simulink model "lateralb747"  (R2024b)
settings: Solver=ode4  StartTime=0.0  StopTime=inf  FixedStep=0.001  RelTol=1e-3
values from neighbouring files (symbols this model uses):
  alpha_init = p.alpharef    [b747lateral.m]
  theta_init = alpha_init    [b747lateral.m]
  V_init = 67.394444    [b747lateral.m]
undefined symbols (not defined in the file or in its folder): p
libraries: simulink_extras x4
settings Model: Creator=adasu  LastModifiedBy=adasu

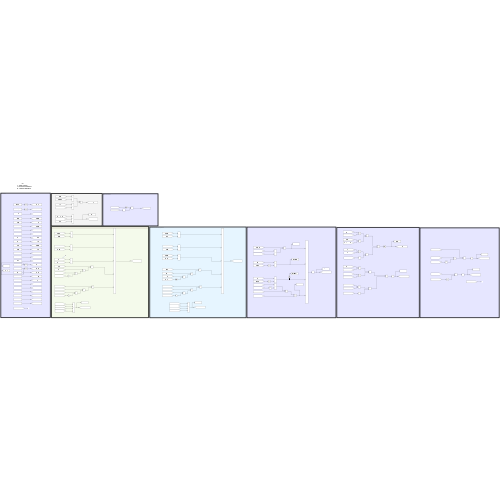
[thumbnail: Simulink's stored preview of the top-level diagram]
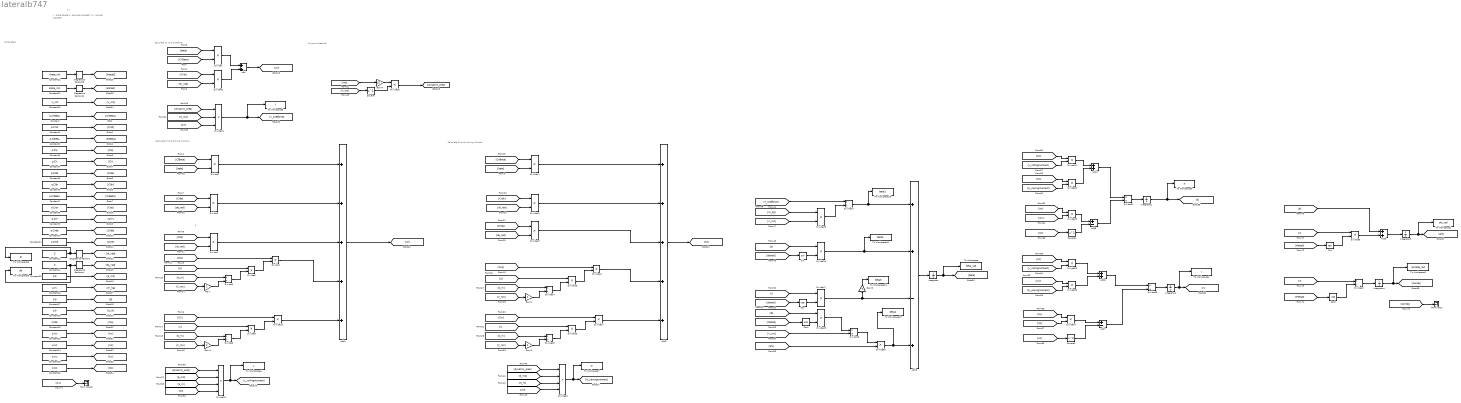
== system lateralb747 ==
  note: Dynamic Pressure
  note: Calculate Cn and Yawing Moment
  note: Calculate Cl and Rolling Moment
  note: Calculate CY and Sideforce
  note: !!!!!
  note: Parameters
  note: Y : SIDE FORCE
      | L : ROLLING MOMENT
      | N : YAWING MOMENT
  note: 0
  Add{,4,6,8} (4 alike) : Sum
  Add1 : Sum  Inputs=5
  Add2 : Sum  Inputs=5
  Add3 : Sum  Inputs=++-+
  Add5 : Sum  Inputs=+-
  Add7 : Sum  Inputs=+-
  Constant : Constant  Value=p.CYBeta
  Constant1 : Constant  Value=p.CYdr
  Constant10 : Constant  Value=p.Cnda
  Constant11 : Constant  Value=p.Cndr
  Constant12 : Constant  Value=5
  Constant14 : Constant  Value=0
  Constant15 : Constant  Value=p.S
  Constant16 : Constant  Value=p.m
  Constant17 : Constant  Value=p.g
  Constant18 : Constant  Value=p.b
  Constant19 : Constant  Value=1.225
  Constant2 : Constant  Value=p.ClBeta
  Constant20 : Constant  Value=V_init
  Constant21 : Constant  Value=alpha_init
  Constant22 : Constant  Value=theta_init
  Constant23 : Constant  Value=p.Ixx
  Constant24 : Constant  Value=p.Ixz
  Constant25 : Constant  Value=p.Iyy
  Constant26 : Constant  Value=p.Izz
  Constant3 : Constant  Value=p.Clp
  Constant4 : Constant  Value=p.Clr
  Constant5 : Constant  Value=p.Clda
  Constant6 : Constant  Value=p.Cldr
  Constant7 : Constant  Value=p.CnBeta
  Constant8 : Constant  Value=p.Cnp
  Constant9 : Constant  Value=p.Cnr
  Cos : Trigonometry  Operator=cos
  Cos1 : Trigonometry  Operator=cos
  Cos2 : Trigonometry  Operator=cos
  Degrees to Radians{,1..3} (4 alike) : simulink_extras/Transformations/Degrees to Radians
  Divide{1..4,6..7,9..13,15..17,19..20,25..28,30..33,35..37,39,41} (29 alike) : Product  Inputs=**
  Divide{5,8,14,18,24,29,34,38,40} (9 alike) : Product  Inputs=*/
  Divide21 : Product  Inputs=***
  Divide22 : Product  Inputs=****
  Divide23 : Product  Inputs=****
  Gain{,1..3} (4 alike) : Gain  Gain=2
  Gain4 : Gain  Gain=1/2
  Gain5 : Gain  Gain=-1
  Integrator{,1..4} (5 alike) : Integrator
  Sin : Trigonometry
  Square : Math  Operator=square
  Square1 : Math  Operator=square
  Square2 : Math  Operator=square
  Tan : Trigonometry  Operator=tan
  Terminator : Terminator
  Terminator2 : Terminator
  To Workspace : ToWorkspace  VariableName=beta_rad  SaveFormat=Timeseries  SampleTime=-1
  To Workspace1 : ToWorkspace  VariableName=phi_rad  SaveFormat=Timeseries  SampleTime=-1
  To Workspace10 : ToWorkspace  VariableName=beta1  SaveFormat=Timeseries  SampleTime=-1
  To Workspace11 : ToWorkspace  VariableName=beta2  SaveFormat=Timeseries  SampleTime=-1
  To Workspace12 : ToWorkspace  VariableName=beta3  SaveFormat=Timeseries  SampleTime=-1
  To Workspace13 : ToWorkspace  VariableName=beta4  SaveFormat=Timeseries  SampleTime=-1
  To Workspace2 : ToWorkspace  VariableName=lambda_rad  SaveFormat=Timeseries  SampleTime=-1
  To Workspace3 : ToWorkspace  VariableName=p  SaveFormat=Timeseries  SampleTime=-1
  To Workspace4 : ToWorkspace  VariableName=r  SaveFormat=Timeseries  SampleTime=-1
  To Workspace5 : ToWorkspace  VariableName=Y  SaveFormat=Timeseries  SampleTime=-1
  To Workspace6 : ToWorkspace  VariableName=L  SaveFormat=Timeseries  SampleTime=-1
  To Workspace7 : ToWorkspace  VariableName=N  SaveFormat=Timeseries  SampleTime=-1
  To Workspace8 : ToWorkspace  VariableName=dr  SaveFormat=Timeseries  SampleTime=-1
  To Workspace9 : ToWorkspace  VariableName=da  SaveFormat=Timeseries  SampleTime=-1
  wires:
  Constant/1 -> [CYBeta]
  Constant1/1 -> [CYdr]
  Constant2/1 -> [ClBeta]
  Constant3/1 -> [Clp]
  Constant4/1 -> [Clr]
  Constant5/1 -> [Clda]
  Constant6/1 -> [Cldr]
  Constant7/1 -> [CnBeta]
  Constant8/1 -> [Cnp]
  Constant9/1 -> [Cnr]
  Constant10/1 -> [Cnda]
  Constant11/1 -> [Cndr]
  Constant12/1 -> To Workspace8/1, Degrees to Radians/1
  Degrees to Radians/1 -> [dr_rad]
  [beta] -> Divide1/1
  [CYBeta] -> Divide1/2
  Divide1/1 -> Add/1
  Divide41/1 -> Add/2
  Add/1 -> [CY]
  Degrees to Radians1/1 -> [da_rad]
  Constant14/1 -> To Workspace9/1, Degrees to Radians1/1
  Constant15/1 -> [S_m2]
  Constant16/1 -> [m_kg]
  Constant17/1 -> [g]
  Constant18/1 -> [b_m]
  Constant19/1 -> [rho]
  Gain4/1 -> Divide20/1
  Divide20/1 -> [dynamic_pres]
  Square/1 -> Divide20/2
  [V_ms] -> Square/1
  [rho] -> Gain4/1
  [S_m2] -> Divide21/2
  [dynamic_pres] -> Divide21/1
  [CY] -> Divide21/3
  Divide21/1 -> To Workspace5/1, [Y_sideforce]
  Divide22/1 -> To Workspace6/1, [L_rollingmoment]
  [dynamic_pres] -> Divide22/1
  [S_m2] -> Divide22/2
  [b_m] -> Divide22/3
  [Cl] -> Divide22/4
  [Cn] -> Divide23/4
  [b_m] -> Divide23/3
  [S_m2] -> Divide23/2
  [dynamic_pres] -> Divide23/1
  Divide23/1 -> To Workspace7/1, [N_yawingmoment]
  [Y_sideforce] -> Divide24/1
  Divide25/1 -> Divide24/2
  Constant21/1 -> Degrees to Radians2/1
  Degrees to Radians2/1 -> [alpha0]
  [alpha0] -> Sin/1
  Sin/1 -> Divide26/2
  [alpha0] -> Cos/1
  Degrees to Radians3/1 -> [theta0]
  Constant22/1 -> Degrees to Radians3/1
  [theta0] -> Cos1/1
  Divide28/1 -> Divide29/1
  [V_ms] -> Divide29/2
  [phi] -> Divide30/2
  Divide29/1 -> Divide30/1
  Divide24/1 -> To Workspace10/1, Add3/1
  Divide26/1 -> To Workspace11/1, Add3/2
  Divide27/1 -> Gain5/1, Add3/3
  Divide30/1 -> To Workspace13/1, Add3/4
  Add3/1 -> Integrator/1
  Integrator/1 -> To Workspace/1, [beta]
  Constant23/1 -> [Ixx]
  Constant24/1 -> [Ixz]
  Constant25/1 -> [Iyy]
  Constant26/1 -> [Izz]
  [Iyy] -> Terminator2/1
  Constant20/1 -> [V_ms]
  [dr_rad] -> Divide41/2
  [CYdr] -> Divide41/1
  [m_kg] -> Divide25/1
  [V_ms] -> Divide25/2
  [p] -> Divide26/1
  Cos/1 -> Divide27/2
  [r] -> Divide27/1
  [g] -> Divide28/1
  Cos1/1 -> Divide28/2
  Gain5/1 -> To Workspace12/1
  Divide3/1 -> Add1/2
  [dr_rad] -> Divide4/2
  [beta] -> Divide2/2
  Divide4/1 -> Add1/3
  [Cldr] -> Divide4/1
  Divide5/1 -> Divide6/2
  Divide9/1 -> Divide10/2
  [r] -> Divide9/1
  Gain/1 -> Divide5/2
  Divide7/1 -> Add1/4
  Divide10/1 -> Add1/5
  [Clr] -> Divide10/1
  Add1/1 -> [Cl]
  [V_ms] -> Gain/1
  [da_rad] -> Divide3/2
  Gain1/1 -> Divide8/2
  [V_ms] -> Gain1/1
  [p] -> Divide6/1
  [b_m] -> Divide5/1
  [ClBeta] -> Divide2/1
  Divide6/1 -> Divide7/2
  Divide8/1 -> Divide9/2
  [Clda] -> Divide3/1
  [b_m] -> Divide8/1
  Divide2/1 -> Add1/1
  [Clp] -> Divide7/1
  Divide18/1 -> Divide19/2
  [V_ms] -> Gain3/1
  Divide19/1 -> Divide17/2
  [r] -> Divide19/1
  Divide12/1 -> Add2/2
  Divide11/1 -> Add2/1
  Divide13/1 -> Add2/3
  Divide16/1 -> Add2/4
  Add2/1 -> [Cn]
  [b_m] -> Divide18/1
  [Cnr] -> Divide17/1
  [b_m] -> Divide14/1
  Gain2/1 -> Divide14/2
  [V_ms] -> Gain2/1
  [p] -> Divide15/1
  Gain3/1 -> Divide18/2
  Divide15/1 -> Divide16/2
  Divide17/1 -> Add2/5
  [Cnp] -> Divide16/1
  Divide14/1 -> Divide15/2
  [CnBeta] -> Divide11/1
  [beta] -> Divide11/2
  [Cndr] -> Divide12/1
  [dr_rad] -> Divide12/2
  [Cnda] -> Divide13/1
  [da_rad] -> Divide13/2
  Divide32/1 -> Add4/2
  Add6/1 -> Divide38/1
  Divide36/1 -> Add6/2
  [N_yawingmoment] -> Divide36/2
  Divide34/1 -> Integrator1/1
  [N_yawingmoment] -> Divide32/2
  [Ixz] -> Divide35/1
  [L_rollingmoment] -> Divide35/2
  [L_rollingmoment] -> Divide31/2
  [Izz] -> Divide31/1
  [Ixx] -> Divide37/1
  [Ixx] -> Divide33/1
  [Izz] -> Divide37/2
  Square2/1 -> Add7/2
  Divide37/1 -> Add7/1
  Divide38/1 -> Integrator2/1
  Add7/1 -> Divide38/2
  Integrator1/1 -> To Workspace3/1, [p]
  [Ixz] -> Divide32/1
  Divide33/1 -> Add5/1
  Divide35/1 -> Add6/1
  [Ixx] -> Divide36/1
  Add5/1 -> Divide34/2
  [Ixz] -> Square1/1
  Divide31/1 -> Add4/1
  [Ixz] -> Square2/1
  Integrator2/1 -> To Workspace4/1, [r]
  [Izz] -> Divide33/2
  Square1/1 -> Add5/2
  Add4/1 -> Divide34/1
  Integrator4/1 -> To Workspace2/1, [lamda]
  Divide40/1 -> Integrator4/1
  [p] -> Add8/1
  [theta0] -> Cos2/1
  Tan/1 -> Divide39/2
  [r] -> Divide40/1
  Integrator3/1 -> To Workspace1/1, [phi]
  [theta0] -> Tan/1
  [lamda] -> Terminator/1
  Cos2/1 -> Divide40/2
  Divide39/1 -> Add8/2
  [r] -> Divide39/1
  Add8/1 -> Integrator3/1
